simulink model "RobotDynamicsControlTest"  (R2026a)
settings: Solver=ode15s  StopTime=2
values from neighbouring files (symbols this model uses):
  action = [0.012 -0.02996 -0.00671 -0.0225 0.003636 -0.01428 gripperAction]    [testRobotDynamicsControl.m]    (also in testRobotPolicy.m = model(image, task))
  scenario = BridgeDataTable    [testRobotDynamicsControl.m]    (also in testUnreal3DAnimation.m)
settings Model: Creator=smaddina  LastModifiedBy=smaddina

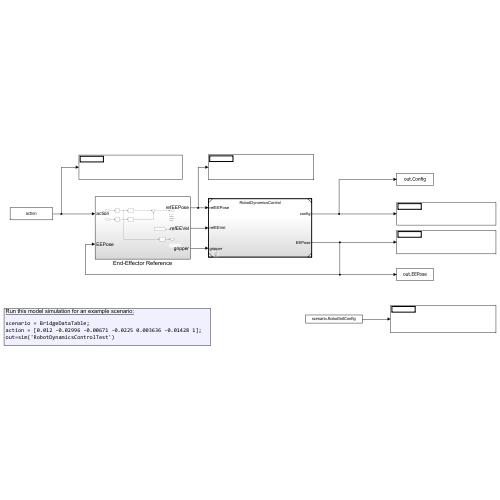
[thumbnail: Simulink's stored preview of the top-level diagram]
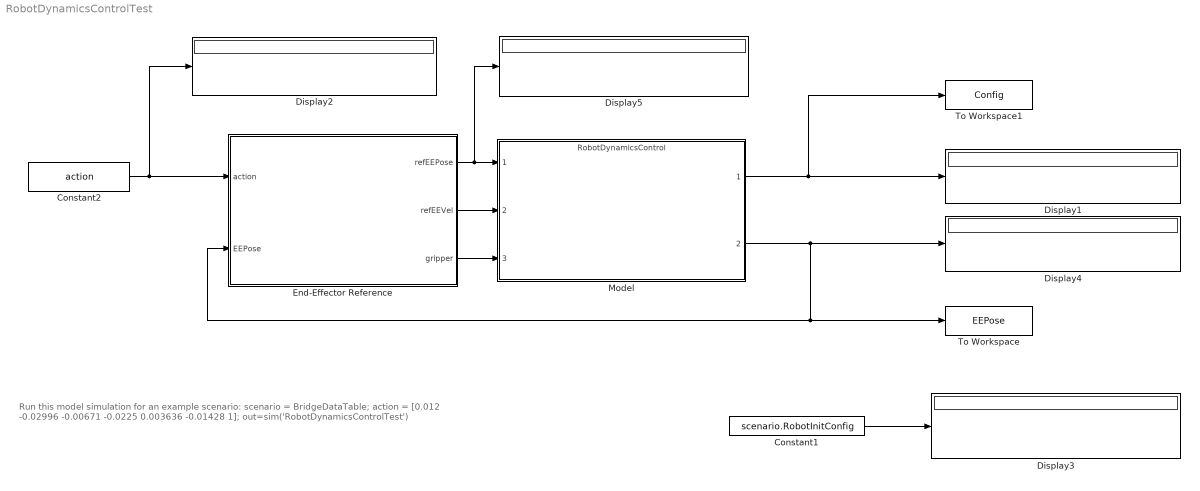
== system RobotDynamicsControlTest ==
  note: Run this model simulation for an example scenario:
      |
      | scenario = BridgeDataTable;
      | action = [0.012 -0.02996 -0.00671 -0.0225 0.003636 -0.01428 1];
      | out=sim('RobotDynamicsControlTest')
  Constant1 : Constant  Value=scenario.RobotInitConfig
  Constant2 : Constant  Value=action  SampleTime=scenario.Ts
  Display{1..5} (5 alike) : Display
  End-Effector Reference : Subsystem
  Model : ModelReference  ModelNameDialog=RobotDynamicsControl.slx  SimulationMode=Normal  ModelReferenceVersion=4.22
  To Workspace : ToWorkspace  VariableName=EEPose  SaveFormat=Timeseries  SampleTime=-1
      settings: MaxDataPoints=1
  To Workspace1 : ToWorkspace  VariableName=Config  SaveFormat=Timeseries  SampleTime=-1
      settings: MaxDataPoints=1
  wires:
  Model/1 -> To Workspace1/1, Display1/1
  Constant1/1 -> Display3/1
  Model/2 -> End-Effector Reference/2(EEPose), To Workspace/1, Display4/1
  Constant2/1 -> Display2/1, End-Effector Reference/1(action)
  End-Effector Reference/1(refEEPose) -> Display5/1, Model/1
  End-Effector Reference/2(refEEVel) -> Model/2
  End-Effector Reference/3(gripper) -> Model/3

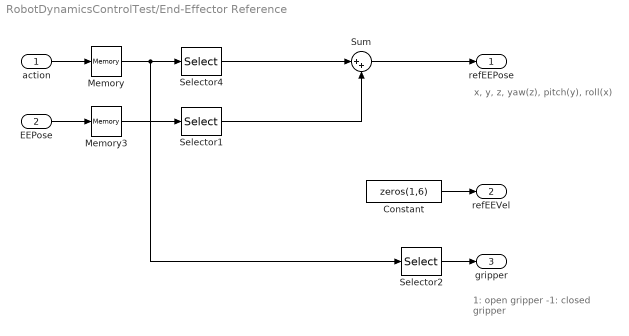
== system RobotDynamicsControlTest/End-Effector Reference ==
  note: x, y, z,
      | yaw(z),
      | pitch(y),
      | roll(x)
  note: 1: open gripper
      | -1: closed gripper
  action : Inport
  EEPose : Inport  Port=2
  Constant : Constant  Value=zeros(1,6)
  Memory : Memory  InitialCondition=[zeros(scenario.NumStates-1,1); 1]  InheritSampleTime=on
  Memory3 : Memory  InitialCondition=scenario.RobotInitState  InheritSampleTime=on
  Selector1 : Selector  InputPortWidth=scenario.NumStates  IndexOptions=Index vector (dialog)  Indices=[1 2 3 4 5 6]  OutputSizes=1
  Selector2 : Selector  InputPortWidth=scenario.NumStates  IndexOptions=Index vector (dialog)  Indices=7  OutputSizes=1
  Selector4 : Selector  InputPortWidth=scenario.NumStates  IndexOptions=Index vector (dialog)  Indices=[1 2 3 4 5 6]  OutputSizes=1
  Sum : Sum  Inputs=|++
  refEEPose : Outport
  refEEVel : Outport  Port=2
  gripper : Outport  Port=3
  wires:
  Sum/1 -> refEEPose/1
  Selector2/1 -> gripper/1
  EEPose/1 -> Memory3/1
  Memory/1 -> Selector4/1, Selector2/1
  action/1 -> Memory/1
  Memory3/1 -> Selector1/1
  Selector4/1 -> Sum/1
  Selector1/1 -> Sum/2
  Constant/1 -> refEEVel/1
